simulink model "testing"  (R2025b)
settings: Solver=FixedStepDiscrete  StartTime=0.0  StopTime=20  RelTol=1e-3
InitFcn:
  | mcb_pmsm_foc_qep_f28379d_SIUnit_data
values from neighbouring files (symbols this model uses):
  A = [ -Rs/L,           0,                  0 ... (first row only)    [mcb_pmsm_fsfb_f28379d_param.m]    (also in v0_pmsm_fsfb_sim_for_flipsky_.m = [; v1_0_3_sim_param_fsfc.m = [)
  inverter = mcb.updateInverterParameters(pmsm,inverter,target)    [mcb_pmsm_foc_qep_f28379d_SIUnit_data.m]
  K = Ka_fsfb(1)    [mcb_pmsm_foc_qep_f28379d_SIUnit_data.m]    (also in mcb_pmsm_fsfb_f28379d_param.m = place(Ai, Bi, desired_poles); v0_pmsm_fsfb_sim_for_flipsky_.m = place(Ai, Bi, desired_poles); v1_0_3_sim_param_fsfc.m = place(Ai, Bi, desired_poles))
  Ki = -Ka_fsfb(2)    [mcb_pmsm_foc_qep_f28379d_SIUnit_data.m]    (also in mcb_pmsm_fsfb_f28379d_param.m = -K(:, n+1:end); v0_pmsm_fsfb_sim_for_flipsky_.m = -K(:, n+1:end); v1_0_3_sim_param_fsfc.m = -K(:, n+1:end))
  lambda_pm = pmsm.FluxPM    [mcb_pmsm_foc_qep_f28379d_SIUnit_data.m]
  PI_params = mcb.calcFOCGains(motor,Ts,Ts_speed,SpdLPFltCoeff=LPFltCoeff)    [mcb_pmsm_foc_qep_f28379d_SIUnit_data.m]
  pmsm = mcb.getPMSMParameters('Teknic2310P')    [mcb_pmsm_foc_qep_f28379d_SIUnit_data.m]
  Speed_Ki_Ts = Kis * Ts_speed    [mcb_pmsm_foc_qep_f28379d_SIUnit_data.m]
  Speed_Kp = Ks    [mcb_pmsm_foc_qep_f28379d_SIUnit_data.m]
  T_pwm = 1/PWM_frequency    (= 5e-05)    [mcb_pmsm_foc_qep_f28379d_SIUnit_data.m]
  target = mcb.getProcessorParameters('F28379D',PWM_frequency)    [mcb_pmsm_foc_qep_f28379d_SIUnit_data.m]
  Ts = T_pwm    (= 5e-05)    [mcb_pmsm_foc_qep_f28379d_SIUnit_data.m]    (also in v0_pmsm_fsfb_sim_for_flipsky_.m = 0.0001; v1_0_3_sim_param_fsfc.m = 0.0001)
  Ts_inverter = T_pwm/2    (= 2.5e-05)    [mcb_pmsm_foc_qep_f28379d_SIUnit_data.m]
  Ts_motor = T_pwm/2    (= 2.5e-05)    [mcb_pmsm_foc_qep_f28379d_SIUnit_data.m]
  Ts_simulink = T_pwm/2    (= 2.5e-05)    [mcb_pmsm_foc_qep_f28379d_SIUnit_data.m]
  Ts_speed = 10*Ts    (= 0.0005)    [mcb_pmsm_foc_qep_f28379d_SIUnit_data.m]
undefined symbols (not defined in the file or in its folder): bit, DiscIntNeverNeededParam, Down, GPTRIP1SEL, GPTRIP2SEL, TZ1, TZ2, Up
libraries: mcbcontrolslib x10, c2802xlib x7, simulink x5, c2837xDlib x4, mcbeeMathTransformLib x3, c280xlib x3, mcbpositiondecoderlib x3, svdschedulerlib x1, autolibpmsmexterior x1, slpidlib x1
(part 1 of 2)
settings Model: SimulationMode=external  ExtModeTrigDuration=8  Creator=LabPC  LastModifiedBy=LabPC
settings OptimizationCC: DefaultUnderspecifiedDataType=single  EnhancedBackFolding=on  PassReuseOutputArgsAs=Individual arguments  MaxStackSize=1024  OptimizeBlockOrder=speed  DifferentSizesBufferReuse=on  OptimizationCustomize=off  EfficientTunableParamExpr=on
settings DebuggingCC: MultiTaskDSMMsg=none  ParameterTunabilityLossMsg=error
settings HardwareCC: ProdBitPerChar=16.0  ProdBitPerInt=16.0  ProdBitPerPointer=32.0  ProdBitPerSizeT=32.0  ProdBitPerPtrDiffT=32.0  ProdLargestAtomicInteger=Integer  ProdLargestAtomicFloat=None  ProdWordSize=16.0  ProdLongLongMode=on  ProdHWDeviceType=Texas Instruments->C2000  HardwareBoardFeatureSet=SoCBlockset
settings SFSimCC: MATLABDynamicMemAlloc=off
settings RTWCC: SystemTargetFile=ert.tlc  HardwareBoard=TI Delfino F28379D LaunchPad  TLCOptions="-aInlineSetEventsForThisBaseRateFcn=TLC_FALSE -aSuppressMultiTaskScheduler=TLC_FALSE   -aRateBasedStepFcn=1"  TemplateMakefile=ert_default_tmf  Toolchain=Texas Instruments Code Composer Studio (C2000)  BuildConfiguration=Faster Runs  CodeProfilingSaveOptions=MetricsOnly  Description=Embedded Coder
settings CodeAppCC: ForceParamTrailComments=on  IgnoreCustomStorageClasses=off  OperatorAnnotations=on  SimulinkDataObjDesc=on  SFDataObjDesc=on  InsertBlockDesc=on
settings ERTTargetCC: ExtModeTransport=4.0  ExtModeStaticAlloc=on  ExtModeAutomaticAllocSize=off  ExtModeStaticAllocSize=10000.0  ExtModeMexFile=ext_xcp  ExtModeIntrfLevel=Level2 - Open  InlinedParameterPlacement=Hierarchical  CodeReplacementLibrary=TI C28x  SupportContinuousTime=on

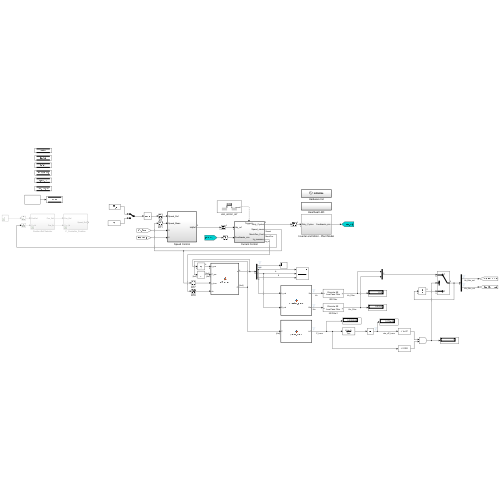
[thumbnail: Simulink's stored preview of the top-level diagram]
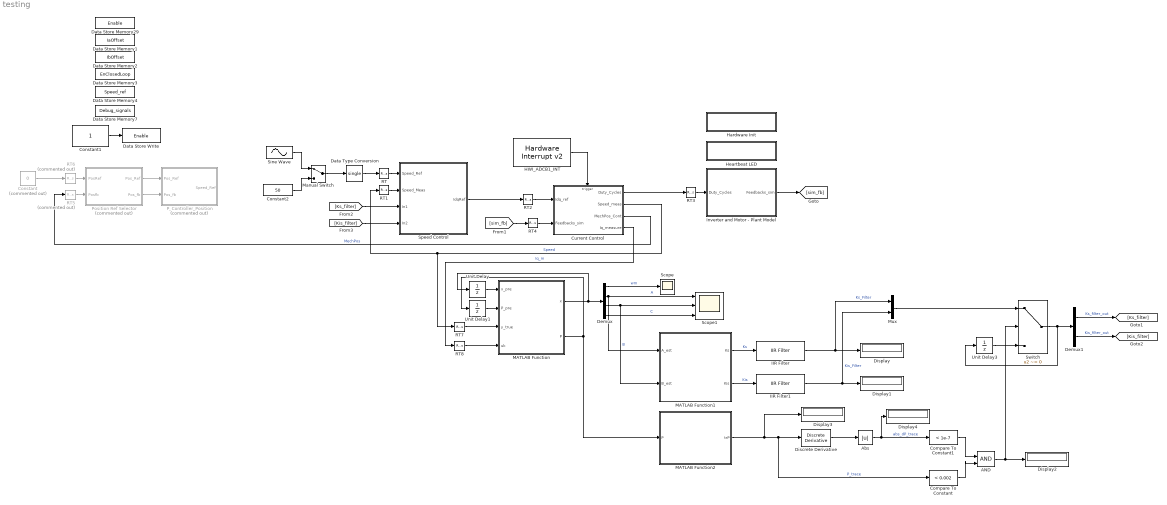
== system testing ==
  AND : Logic  IconShape=distinctive  AllPortsSameDT=off  OutDataTypeStr=boolean
  Abs : Abs  SaturateOnIntegerOverflow=off
  Compare To Constant : simulink/Logic and Bit Operations/Compare To Constant  relop=<  const=0.002  OutDataTypeStr=boolean
  Compare To Constant1 : simulink/Logic and Bit Operations/Compare To Constant  relop=<  const=1e-7  OutDataTypeStr=boolean
  Constant : Constant  Commented=on  Value=0
  Constant1 : Constant  OutDataTypeStr=boolean
  Constant2 : Constant  Value=50
  Current Control : Subsystem
      settings: RTWSystemCode=Nonreusable function
  Data Store Memory1 : DataStoreMemory  DataStoreName=IaOffset  InitialValue=inverter.CtSensAOffset  ShowAdditionalParam=off
  Data Store Memory2 : DataStoreMemory  DataStoreName=IbOffset  InitialValue=inverter.CtSensBOffset  ShowAdditionalParam=off
  Data Store Memory29 : DataStoreMemory  DataStoreName=Enable  ShowAdditionalParam=off  OutDataTypeStr=boolean
  Data Store Memory3 : DataStoreMemory  DataStoreName=EnClosedLoop  ShowAdditionalParam=off  OutDataTypeStr=boolean
  Data Store Memory4 : DataStoreMemory  DataStoreName=Speed_ref  ShowAdditionalParam=off  OutDataTypeStr=dataType
  Data Store Memory7 : DataStoreMemory  DataStoreName=Debug_signals  InitialValue=5  ShowAdditionalParam=off  OutDataTypeStr=uint16
  Data Store Write : DataStoreWrite  DataStoreName=Enable  IndexOptions=Index vector (dialog)  Indices=1  OutputSizes=1
  Data Type Conversion : DataTypeConversion  OutDataTypeStr=single  SaturateOnIntegerOverflow=off  RndMeth=Floor
  Demux : Demux
  Demux1 : Demux  Outputs=2
  Discrete Derivative : simulink/Discrete/Discrete Derivative  gainval=1.0  ICPrevScaledInput=10  OutMin=[]  OutMax=[]  OutDataType=fixdt(1, 16)  OutScaling=2^-10  DoSatur=off
  Display{,1..4} (5 alike) : Display
  HWI_ADCB1_INT : svdschedulerlib/Hardware Interrupt v2  ISRGroup=ADC - Analog to Digital Converter  ISRName=ADCA1_INT  ISRNumber=32  NumEventsToServe=1  EventsList={'on','EOC event','1';'off','Overflow event','2';'off','Custom event','3'}  SelectedEvents={'event1'}  TaskPriority=30  DisablePreemption=off  ClearInterruptFlagsAtEndOfEvent=on  InterruptDefinitionFile=$(TARGET_ROOT)/registry/interrupts/F2837xS_interrupts.xml  HardwareBoard=F2837x  EnableSimPort=off
      settings: LibrarySourceBlock=c2000lib/Scheduling/Hardware Interrupt
  Hardware Init : Subsystem  TreatAsAtomicUnit=on
  Heartbeat LED : Subsystem  TreatAsAtomicUnit=on
  IIR Filter : mcbcontrolslib/IIR Filter  VariantControl=Low Pass Filter  VariantSelect=Low-pass  FilterConstantInputType=Specify via dialog  Filter_constant=0.001  InitialOutput=Specify via dialog  InitialOutputValue=0  ExternalReset=none  advancedSettings=off  Ts=50e-6  cutOff_freq=3.1863
  IIR Filter1 : mcbcontrolslib/IIR Filter  VariantControl=Low Pass Filter  VariantSelect=Low-pass  FilterConstantInputType=Specify via dialog  Filter_constant=0.001  InitialOutput=Specify via dialog  InitialOutputValue=0  ExternalReset=none  advancedSettings=off  Ts=50e-6  cutOff_freq=3.1863
  Inverter and Motor - Plant Model : Subsystem
  MATLAB Function : MATLAB Function  TreatAsAtomicUnit=on
  MATLAB Function1 : MATLAB Function  TreatAsAtomicUnit=on
  MATLAB Function2 : MATLAB Function  TreatAsAtomicUnit=on
  Manual Switch : ManualSwitch
  Mux : Mux  Inputs=2
  P_Controller_Position : Subsystem  Commented=on
  Position Ref Selector : Subsystem  Commented=on
  RT{,1,7..8} (4 alike) : RateTransition  Deterministic=off  OutPortSampleTime=Ts_speed
  RT2 : RateTransition  Deterministic=off
  RT3 : RateTransition  Deterministic=off
  RT4 : RateTransition  Deterministic=off
  RT5 : RateTransition  Commented=on  Deterministic=off  OutPortSampleTime=Ts_speed
  RT6 : RateTransition  Commented=on  Deterministic=off  OutPortSampleTime=Ts_speed
  Scope : Scope
      settings: ActiveDisplayYMinimum=-2525.7371063232422  ActiveDisplayYMaximum=2611.2176971435547
  Scope1 : Scope  NumInputPorts=3
      settings: ActiveDisplayYMinimum=-2525.7371063232422  ActiveDisplayYMaximum=2611.2176971435547
  Sine Wave : Sin  Amplitude=100  Frequency=5  SampleTime=Ts_speed
  Speed Control : Subsystem  TreatAsAtomicUnit=on  SystemSampleTime=Ts_speed
  Switch : Switch  Criteria=u2 ~= 0  SaturateOnIntegerOverflow=off  InputSameDT=off
  Unit Delay : UnitDelay  InitialCondition=[0; 0.3734; 5438; 0.1]  SampleTime=-1  HasFrameUpgradeWarning=on
  Unit Delay1 : UnitDelay  InitialCondition=diag([1 10 10 100])  SampleTime=-1  HasFrameUpgradeWarning=on
  Unit Delay3 : UnitDelay  InitialCondition=[0.0202, 2.7604e-04]  SampleTime=-1  HasFrameUpgradeWarning=on
  wires:
  RT4/1 -> Current Control/2(Feedbacks_sim)
  Speed Control/1(IdqRef) -> RT2/1
  Inverter and Motor - Plant Model/1(Feedbacks_sim) -> [sim_fb]
  Current Control/1(Duty_Cycles) -> RT3/1
  Current Control/2(Speed_meas) -> RT1/1, RT7/1  "Speed"
  RT/1 -> Speed Control/1(Speed_Ref)
  RT2/1 -> Current Control/1(Idq_ref)
  RT1/1 -> Speed Control/2(Speed_Meas)
  RT3/1 -> Inverter and Motor - Plant Model/1(Duty_Cycles)
  [sim_fb] -> RT4/1
  Constant1/1 -> Data Store Write/1
  HWI_ADCB1_INT/1 -> Current Control/Trigger
  Constant/1 -> RT6/1
  Position Ref Selector/1(Pos_Ref) -> P_Controller_Position/1(Pos_Ref)
  Position Ref Selector/2(Pos_fb) -> P_Controller_Position/2(Pos_fb)
  Current Control/3(MechPos_Cont) -> RT5/1  "MechPos"
  RT5/1 -> Position Ref Selector/2(Posfb)
  RT6/1 -> Position Ref Selector/1(PosRef)
  MATLAB Function/1(x) -> Demux/1, Unit Delay/1
  Unit Delay/1 -> MATLAB Function/1(x_pre)
  Unit Delay1/1 -> MATLAB Function/2(P_pre)
  MATLAB Function/2(P) -> MATLAB Function2/1(P), Unit Delay1/1
  RT7/1 -> MATLAB Function/3(y_true)
  Current Control/4(Iq_measure) -> RT8/1  "Iq_m"
  RT8/1 -> MATLAB Function/4(uk)
  Demux/3 -> MATLAB Function1/2(B_est), Scope1/2  "B"
  Demux/2 -> MATLAB Function1/1(A_est), Scope1/1  "A"
  Data Type Conversion/1 -> RT/1
  MATLAB Function1/1(Ks) -> IIR Filter/1  "Ks"
  IIR Filter/1 -> Mux/1, Display/1  "Ks_Filter"
  MATLAB Function1/2(Kis) -> IIR Filter1/1  "Kis"
  IIR Filter1/1 -> Mux/2, Display1/1  "Kis_Filter"
  Manual Switch/1 -> Data Type Conversion/1
  Sine Wave/1 -> Manual Switch/1
  Constant2/1 -> Manual Switch/2
  MATLAB Function2/1(trP) -> Display3/1, Discrete Derivative/1, Compare To Constant/1  "P_trace"
  Discrete Derivative/1 -> Abs/1
  Abs/1 -> Display4/1, Compare To Constant1/1  "abs_dP_trace"
  Compare To Constant1/1 -> AND/1
  Compare To Constant/1 -> AND/2
  AND/1 -> Display2/1, Switch/2
  Mux/1 -> Switch/1
  Unit Delay3/1 -> Switch/3
  Switch/1 -> Unit Delay3/1, Demux1/1
  Demux1/1 -> [Ks_filter]  "Ks_filter_out"
  Demux1/2 -> [Kis_filter]  "Kis_filter_out"
  [Ks_filter] -> Speed Control/3(In1)
  [Kis_filter] -> Speed Control/4(In2)
  Demux/1 -> Scope/1  "wm"
  Demux/4 -> Scope1/3  "C"

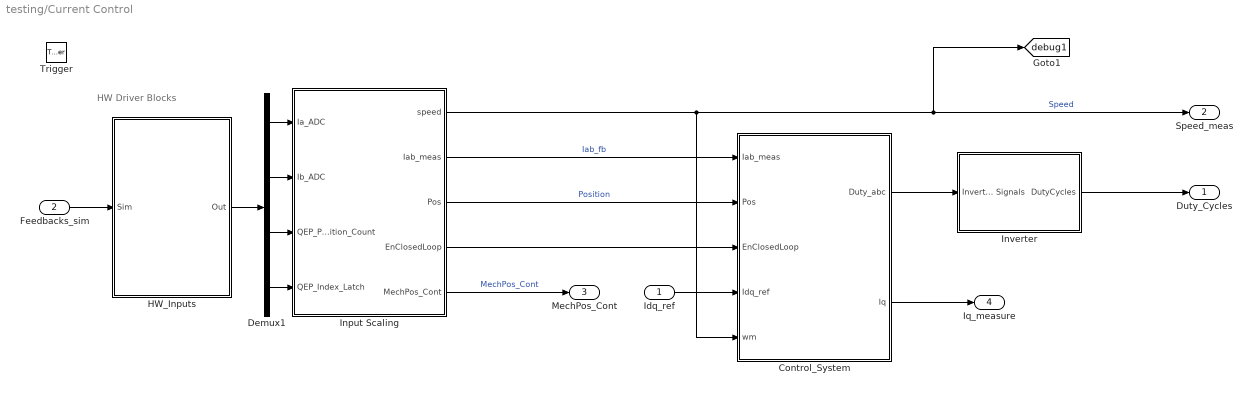
== system testing/Current Control ==
  note: HW Driver Blocks
  Idq_ref : Inport
  Feedbacks_sim : Inport  Port=2
  Trigger : TriggerPort  TriggerType=function-call  VariantControl=Variant  PortDimensions=1
  Control_System : Subsystem  TreatAsAtomicUnit=on
  Demux1 : Demux
  HW_Inputs : Subsystem  Variant=on  VariantControlMode=sim codegen switching
  Input Scaling : Subsystem
  Inverter : Subsystem  Variant=on  VariantControlMode=sim codegen switching
  Duty_Cycles : Outport  InitialOutput=0  VectorParamsAs1DForOutWhenUnconnected=off
  Speed_meas : Outport  Port=2  InitialOutput=0  VectorParamsAs1DForOutWhenUnconnected=off
  MechPos_Cont : Outport  Port=3  InitialOutput=0  VectorParamsAs1DForOutWhenUnconnected=off
  Iq_measure : Outport  Port=4  InitialOutput=0  VectorParamsAs1DForOutWhenUnconnected=off
  tag scope: debug1=global
  wires:
  Input Scaling/3(Pos) -> Control_System/2(Pos)  "Position"
  Idq_ref/1 -> Control_System/4(Idq_ref)
  Input Scaling/1(speed) -> Control_System/5(wm), Speed_meas/1, [debug1]  "Speed"
  Input Scaling/2(Iab_meas) -> Control_System/1(Iab_meas)  "Iab_fb"
  Demux1/1 -> Input Scaling/1(Ia_ADC)
  Demux1/2 -> Input Scaling/2(Ib_ADC)
  Demux1/3 -> Input Scaling/3(QEP_Position_Count)
  Demux1/4 -> Input Scaling/4(QEP_Index_Latch)
  Inverter/1(DutyCycles) -> Duty_Cycles/1
  HW_Inputs/1(Out) -> Demux1/1
  Feedbacks_sim/1 -> HW_Inputs/1(Sim)
  Input Scaling/4(EnClosedLoop) -> Control_System/3(EnClosedLoop)
  Control_System/1(Duty_abc) -> Inverter/1(Inverter Signals)
  Input Scaling/5(MechPos_Cont) -> MechPos_Cont/1  "MechPos_Cont"
  Control_System/2(Iq) -> Iq_measure/1

== system testing/Hardware Init ==
  6PWM_Mode : Constant  Priority=1000  Value=0x3A16  OutDataTypeStr=uint16  SampleTime=-1
  ADC_Gain_Setting : Constant  Priority=1000  Value=inverter.SPI_Gain_Setting  OutDataTypeStr=uint16  SampleTime=-1
  Event Listener : EventListener  DisableCoverage=on  EventName=reset
  Mux : Mux  Inputs=2
  Variant Subsystem : Subsystem  Variant=on  VariantControlMode=sim codegen switching
  wires:
  6PWM_Mode/1 -> Mux/1
  ADC_Gain_Setting/1 -> Mux/2
  Mux/1 -> Variant Subsystem/1(In1)

== system testing/Heartbeat LED ==
  note: Heartbeat LED 1HZ
  Heartbeat LED : Subsystem  Variant=on  VariantControlMode=sim codegen switching
  RED_LED : Constant  OutDataTypeStr=uint16  SampleTime=2
  wires:
  RED_LED/1 -> Heartbeat LED/1(In1)

== system testing/Inverter and Motor - Plant Model ==
  Duty_Cycles : Inport
  Codegeneration : Subsystem
  Simulation : Subsystem
  Variant Sink : VariantSink  VariantControlMode=sim codegen switching  VariantControls={(codegen), (sim)}
  Variant Source1 : VariantSource  VariantControlMode=sim codegen switching  VariantControls={(codegen), (sim)}
  Feedbacks_sim : Outport  VectorParamsAs1DForOutWhenUnconnected=off
  wires:
  Variant Source1/1 -> Feedbacks_sim/1
  Simulation/1(Feedbacks) -> Variant Source1/2
  Codegeneration/1(Feedbacks) -> Variant Source1/1
  Duty_Cycles/1 -> Variant Sink/1
  Variant Sink/2 -> Simulation/1(Duty_Cycles)
  Variant Sink/1 -> Codegeneration/1(Duty_Cycles)

== system testing/P_Controller_Position ==
  Pos_Ref : Inport
  Pos_fb : Inport  Port=2
  Constant : Constant  Value=10  OutDataTypeStr=dataType
  Divide : Product  Inputs=**  OutDataTypeStr=dataType  RndMeth=Simplest
  Saturation : Saturate  UpperLimit=5000  LowerLimit=-5000
  Sum : Sum  Inputs=|+-  OutDataTypeStr=Inherit: Same as first input
  Speed_Ref : Outport
  wires:
  Constant/1 -> Divide/2
  Saturation/1 -> Speed_Ref/1
  Divide/1 -> Saturation/1
  Pos_Ref/1 -> Sum/1
  Pos_fb/1 -> Sum/2
  Sum/1 -> Divide/1  "error_pos"

== system testing/Position Ref Selector ==
  PosRef : Inport
  Posfb : Inport  Port=2
  AND : Logic  IconShape=distinctive  AllPortsSameDT=off  OutDataTypeStr=boolean
  Data Store Read : DataStoreRead  DataStoreName=EnClosedLoop  IndexOptions=Index vector (dialog)  Indices=1  OutputSizes=1
  Data Store Read1 : DataStoreRead  DataStoreName=Enable  IndexOptions=Index vector (dialog)  Indices=1  OutputSizes=1
  Switch : Switch  Criteria=u2 > Threshold  SaturateOnIntegerOverflow=off  InputSameDT=off
  Pos_Ref : Outport
  Pos_fb : Outport  Port=2
  wires:
  Data Store Read/1 -> AND/1
  AND/1 -> Switch/2
  PosRef/1 -> Switch/1
  Data Store Read1/1 -> AND/2
  Switch/1 -> Pos_Ref/1
  Posfb/1 -> Pos_fb/1, Switch/3

== system testing/Speed Control ==
  Speed_Ref : Inport
  Speed_Meas : Inport  Port=2
  In1 : Inport  Port=3
  In2 : Inport  Port=4
  Id_ref : Constant  Value=0  OutDataTypeStr=dataType  SampleTime=Ts_speed
  Mux1 : Mux  Inputs=2
  PI_Controller_Speed : Subsystem
  Subsystem : Subsystem
  IdqRef : Outport  VectorParamsAs1DForOutWhenUnconnected=off
  wires:
  Speed_Meas/1 -> PI_Controller_Speed/2(N_fb), Subsystem/2(Speed_Ref_Open)  "Speed_fb"
  Subsystem/1(Speed_Ref_PU) -> PI_Controller_Speed/1(N_ref)  "Speed_Ref"
  Id_ref/1 -> Mux1/1
  PI_Controller_Speed/1(Iq_ref) -> Mux1/2
  Mux1/1 -> IdqRef/1
  Speed_Ref/1 -> Subsystem/1(Speed_Ref_In)
  In1/1 -> PI_Controller_Speed/3(In1)  "Ks_filter"
  In2/1 -> PI_Controller_Speed/4(In2)  "Kis_filter"

== system testing/Current Control/Control_System ==
  Iab_meas : Inport
  Pos : Inport  Port=2
  EnClosedLoop : Inport  Port=3
  Idq_ref : Inport  Port=4
  wm : Inport  Port=5
  Closed Loop Control : Subsystem
  NOT : Logic  Operator=NOT  IconShape=distinctive  AllPortsSameDT=off  OutDataTypeStr=boolean
  Open Loop Start-Up : Subsystem
  Switch4 : Switch  Threshold=0.5  OutDataTypeStr=Inherit: Inherit via back propagation  RndMeth=Simplest  SaturateOnIntegerOverflow=off  InputSameDT=off
  Duty_abc : Outport  VectorParamsAs1DForOutWhenUnconnected=off
  Iq : Outport  Port=2  VectorParamsAs1DForOutWhenUnconnected=off
  wires:
  EnClosedLoop/1 -> NOT/1, Switch4/2, Closed Loop Control/Enable
  Open Loop Start-Up/1(Duty_abc) -> Switch4/3
  Iab_meas/1 -> Closed Loop Control/1(Iab_meas)
  Pos/1 -> Closed Loop Control/2(Pos)
  Idq_ref/1 -> Closed Loop Control/3(Idq_ref)
  Closed Loop Control/2(Duty_abc) -> Switch4/1
  NOT/1 -> Open Loop Start-Up/Enable
  Switch4/1 -> Duty_abc/1  "PWM_Duty_Cycles"
  Closed Loop Control/1(Iq) -> Iq/1
  wm/1 -> Closed Loop Control/4(wm)

== system testing/Current Control/HW_Inputs ==
  Sim : Inport
  Sensor Driver Blocks (codegen) : Subsystem  VariantControl=(codegen)
  Sensor Driver Blocks (sim) : Subsystem  VariantControl=(sim)
  Out : Outport

== system testing/Current Control/Input Scaling ==
  note: Current Measurements
  note: Position & Speed Measurements
  note: QEP
  Ia_ADC : Inport
  Ib_ADC : Inport  Port=2
  QEP_Position_Count : Inport  Port=3
  QEP_Index_Latch : Inport  Port=4
  " Calculate Position and Speed" : Subsystem
  Calculate Phase Currents : Subsystem
  IndexOffset : Constant  Value=pmsm.PositionOffset * 2 * pi  OutDataTypeStr=dataType  SampleTime=-1
  speed : Outport
  Iab_meas : Outport  Port=2
  Pos : Outport  Port=3
  EnClosedLoop : Outport  Port=4
  MechPos_Cont : Outport  Port=5
  wires:
  " Calculate Position and Speed"/2(speed) -> speed/1
  Calculate Phase Currents/1(Iab_meas) -> Iab_meas/1  "Iab_fb"
  QEP_Position_Count/1 -> " Calculate Position and Speed"/1(QEP_Position_Count)
  " Calculate Position and Speed"/1(Theta_e) -> Pos/1
  Ia_ADC/1 -> Calculate Phase Currents/1(Ia_ADC)
  Ib_ADC/1 -> Calculate Phase Currents/2(Ib_ADC)
  QEP_Index_Latch/1 -> " Calculate Position and Speed"/2(QEP_Index_Latch)
  IndexOffset/1 -> " Calculate Position and Speed"/3(Offset)
  " Calculate Position and Speed"/3(IndexFound) -> EnClosedLoop/1
  " Calculate Position and Speed"/4(MechPos_Cont) -> MechPos_Cont/1

== system testing/Current Control/Inverter ==
  Inverter Signals : Inport
  Code Generation : Subsystem  VariantControl=(codegen)
  Simulation : Subsystem  VariantControl=(sim)
  DutyCycles : Outport  VectorParamsAs1DForOutWhenUnconnected=off

== system testing/Hardware Init/Variant Subsystem ==
  In1 : Inport
  Code Generation : Subsystem  VariantControl=(codegen)
  Simulation : Subsystem  VariantControl=(sim)

== system testing/Heartbeat LED/Heartbeat LED ==
  In1 : Inport
  Code generation : Subsystem  VariantControl=(codegen)
  Simulation : Subsystem  VariantControl=(sim)

== system testing/Inverter and Motor - Plant Model/Codegeneration ==
  Duty_Cycles : Inport
  Ground : Ground
  Terminator : Terminator
  Feedbacks : Outport  VectorParamsAs1DForOutWhenUnconnected=off
  wires:
  Duty_Cycles/1 -> Terminator/1
  Ground/1 -> Feedbacks/1

== system testing/Inverter and Motor - Plant Model/Simulation ==
  Duty_Cycles : Inport
  Inverter : Subsystem
  Load_Profile (Torque) : Subsystem
  RT1 : RateTransition  Deterministic=off  OutPortSampleTime=Ts_simulink
  RT3 : RateTransition  Deterministic=off  OutPortSampleTime=Ts_simulink
  Rate Transition : RateTransition  Integrity=off  OutPortSampleTime=Ts_motor
  Rate Transition1 : RateTransition  Integrity=off  OutPortSampleTime=Ts_motor
  Sensor_Measurements : Subsystem
  Surface Mount PMSM : autolibpmsmexterior/Surface Mount PMSM  port_config=Torque  sim_type=Discrete  Ts=Ts_motor  P=pmsm.p  Rs=pmsm.Rs + inverter.R_board  Ldq_=pmsm.Ld  KConstText=Permanent flux linkage constant (lambda_pm):  lambda_pm=pmsm.FluxPM  Ke=159.9771  Kt=1.323  mechanical=[pmsm.J, pmsm.B, 0]  idq0=[0 0]  theta_init=0  omega_init=0  KConst=pmsm.FluxPM  lambda_pm_calc=pmsm.FluxPM  RefBlkName='autolibpmsmexterior/Surface Mount PMSM'  aMode=5  Ldq="[0.00105     0.00105]"
  Terminator : Terminator
  Feedbacks : Outport  VectorParamsAs1DForOutWhenUnconnected=off
  wires:
  Rate Transition1/1 -> Surface Mount PMSM/1
  Surface Mount PMSM/2 -> RT1/1  "Iabc"
  Surface Mount PMSM/3 -> Terminator/1
  Rate Transition/1 -> Surface Mount PMSM/2  "PhaseVoltage"
  RT1/1 -> Sensor_Measurements/2(PhaseCurr)
  Duty_Cycles/1 -> Inverter/1(Duty_abc)
  Inverter/1(Vabc) -> Rate Transition/1
  RT3/1 -> Sensor_Measurements/1(Info)
  Surface Mount PMSM/1 -> RT3/1
  Load_Profile (Torque)/1(Load_Trq) -> Rate Transition1/1
  Sensor_Measurements/1(Sim_fb) -> Feedbacks/1

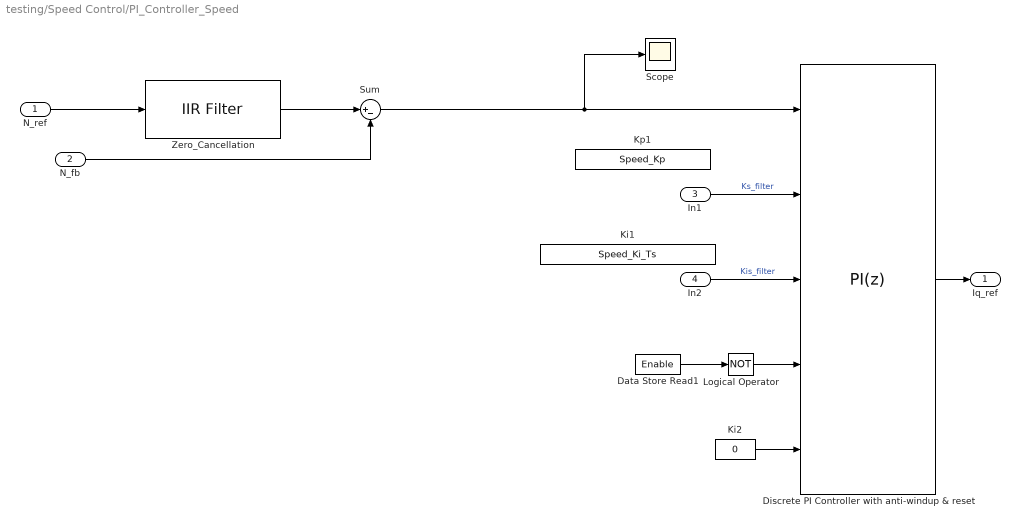
== system testing/Speed Control/PI_Controller_Speed ==
  N_ref : Inport
  N_fb : Inport  Port=2
  In1 : Inport  Port=3
  In2 : Inport  Port=4
  Data Store Read1 : DataStoreRead  DataStoreName=Enable  IndexOptions=Index vector (dialog)  Indices=1  OutputSizes=1
  Discrete PI Controller with anti-windup & reset : slpidlib/PID Controller  Controller=PI  Form=Parallel  TimeDomain=Discrete-time  UseExternalTs=off  SampleTime=-1  IntegratorMethod=Forward Euler  FilterMethod=Forward Euler  ControllerParametersSource=external  P=1  I=1  UseKiTs=on  D=0  UseExternalDerivativeSource=off  N=100  UseFilter=on  TunerSelectOption=Transfer Function Based (PID Tuner App)  InitialConditionSource=external  InitialConditionForIntegrator=0  InitialConditionForFilter=0  DifferentiatorICPrevScaledInput=0  ExternalReset=level  TrackingMode=off  Kt=1  LimitOutput=on  SatLimitsSource=internal  UpperSaturationLimit=inverter.ISenseMax  LowerSaturationLimit=-inverter.ISenseMax  LinearizeAsGain=on  AntiWindupMode=clamping  Kb=1  LimitIntegrator=off  UpperIntegratorSaturationLimit=inf  LowerIntegratorSaturationLimit=-inf  RndMeth=Simplest  POutMin=[]  POutMax=[]  IOutMin=[]  IOutMax=[]  DOutMin=[]  DOutMax=[]  NOutMin=[]  NOutMax=[]  SumOutMin=[]  SumOutMax=[]  SaturationOutDataTypeStr=Inherit: Inherit via back propagation  SaturationOutMin=[]  SaturationOutMax=[]  PParamMin=[]  PParamMax=[]  IParamMin=[]  IParamMax=[]  DParamMin=[]  DParamMax=[]  NParamMin=[]  NParamMax=[]  KbParamMin=[]  KbParamMax=[]  KtParamMin=[]  KtParamMax=[]  KbOutMin=[]  KbOutMax=[]  KtOutMin=[]  KtOutMax=[]  IntegratorOutMin=[]  IntegratorOutMax=[]  FilterOutMin=[]  FilterOutMax=[]  SumI1OutMin=[]  SumI1OutMax=[]  SumI2OutMin=[]  SumI2OutMax=[]  SumI3OutMin=[]  SumI3OutMax=[]  SumI4OutMin=[]  SumI4OutMax=[]  SumDOutMin=[]  SumDOutMax=[]  DifferentiatorOutMin=[]  DifferentiatorOutMax=[]  FilterDiffOutCoefMin=[]  FilterDiffOutCoefMax=[]  ReciprocalOutMin=[]  ReciprocalOutMax=[]  SumDenOutMin=[]  SumDenOutMax=[]  SumNumOutMin=[]  SumNumOutMax=[]  DivideOutMin=[]  DivideOutMax=[]  UdiffTsProdOutMin=[]  UdiffTsProdOutMax=[]  NTsProdOutMin=[]  NTsProdOutMax=[]  UintegralTsProdOutMin=[]  UintegralTsProdOutMax=[]  UngainTsProdOutMin=[]  UngainTsProdOutMax=[]  ClampingZeroOutDataTypeStr=Inherit: Inherit via back propagation  ClampingZeroOutMin=[]  ClampingZeroOutMax=[]  FilterDenConstantOutDataTypeStr=Inherit: Inherit via back propagation  FilterDenConstantOutMin=[]  FilterDenConstantOutMax=[]  PCopyOutDataTypeStr=Inherit: Inherit via back propagation  PCopyOutMin=[]  PCopyOutMax=[]  NCopyOutDataTypeStr=Inherit: Inherit via back propagation  NCopyOutMin=[]  NCopyOutMax=[]  IntegratorContinuousStateAttributes=''  IntegratorStateMustResolveToSignalObject=off  IntegratorRTWStateStorageClass=Auto  FilterContinuousStateAttributes=''  FilterStateMustResolveToSignalObject=off  FilterRTWStateStorageClass=Auto  ParallelPVariant=ExternalParameters  IdealPVariant=Disabled  IVariant=ExternalParameters  DVariant=Disabled  IntegratorVariant=Discrete  SatVariant=Enabled  AWVariant=DiscClampingParallel  PCopyVariant=Disabled  TRVariant=Disabled  FdbkBlocksVariant=Forward  IdealPFdbkVariant=Disabled  SatFdbkVariant=Disabled  DerivativeFilterVariant=Disabled  NVariant=Disabled  NCopyVariant=Disabled_SignalSpec  FilterICVariant=Disabled  IntegratorICVariant=ExternalICs  ExternalResetVariant=ExternalReset  TRSumVariant=Passthrough  SumFdbkVariant=Disabled  SumVariant=Sum_PI  TsampFilterVariant=InternalTs  TsampNgainVariant=Passthrough  TsampIntegralVariant=Disabled_SignalSpec  ExternalSaturationOutDataTypeStr=Inherit: Same as second input  DerivativeSourceVariant=Disabled  PreIntVariant=InternalPreInt
      settings: LibrarySourceBlock=mcbcontrolslib/PI Controller
  Ki1 : Constant  Value=Speed_Ki_Ts  OutDataTypeStr=dataType  SampleTime=-1
  Ki2 : Constant  Value=0  OutDataTypeStr=dataType  SampleTime=-1
  Kp1 : Constant  Value=Speed_Kp  OutDataTypeStr=dataType  SampleTime=-1
  Logical Operator : Logic  Operator=NOT  IconShape=distinctive  AllPortsSameDT=off  OutDataTypeStr=boolean
  Scope : Scope
      settings: ActiveDisplayYMinimum=-12.100083367889781  ActiveDisplayYMaximum=11.106556656295403  DataLoggingVariableName=ScopeData7
  Sum : Sum  Inputs=|+-  OutDataTypeStr=Inherit: Same as first input
  Zero_Cancellation : mcbcontrolslib/IIR Filter  VariantControl=Low Pass Filter  VariantSelect=Low-pass  FilterConstantInputType=Specify via dialog  Filter_constant=0.01*(Ts_speed/Ts)  InitialOutput=Specify via dialog  InitialOutputValue=0  ExternalReset=none  advancedSettings=off  Ts=50e-6  cutOff_freq=353.6777
  Iq_ref : Outport  VectorParamsAs1DForOutWhenUnconnected=off
  wires:
  Discrete PI Controller with anti-windup & reset/1 -> Iq_ref/1
  Sum/1 -> Scope/1, Discrete PI Controller with anti-windup & reset/1
  Logical Operator/1 -> Discrete PI Controller with anti-windup & reset/4
  Ki2/1 -> Discrete PI Controller with anti-windup & reset/5
  Data Store Read1/1 -> Logical Operator/1
  N_ref/1 -> Zero_Cancellation/1
  N_fb/1 -> Sum/2
  Zero_Cancellation/1 -> Sum/1
  In1/1 -> Discrete PI Controller with anti-windup & reset/2  "Ks_filter"
  In2/1 -> Discrete PI Controller with anti-windup & reset/3  "Kis_filter"

== system testing/Speed Control/Subsystem ==
  Speed_Ref_In : Inport
  Speed_Ref_Open : Inport  Port=2
  AND : Logic  IconShape=distinctive  AllPortsSameDT=off  OutDataTypeStr=boolean
  Data Store Read : DataStoreRead  DataStoreName=EnClosedLoop  IndexOptions=Index vector (dialog)  Indices=1  OutputSizes=1
  Data Store Read1 : DataStoreRead  DataStoreName=Enable  IndexOptions=Index vector (dialog)  Indices=1  OutputSizes=1
  Switch : Switch  Criteria=u2 > Threshold  Threshold=0.5  SaturateOnIntegerOverflow=off  InputSameDT=off
  Speed_Ref_PU : Outport
  wires:
  Switch/1 -> Speed_Ref_PU/1
  Speed_Ref_Open/1 -> Switch/3
  Speed_Ref_In/1 -> Switch/1
  AND/1 -> Switch/2
  Data Store Read/1 -> AND/1
  Data Store Read1/1 -> AND/2

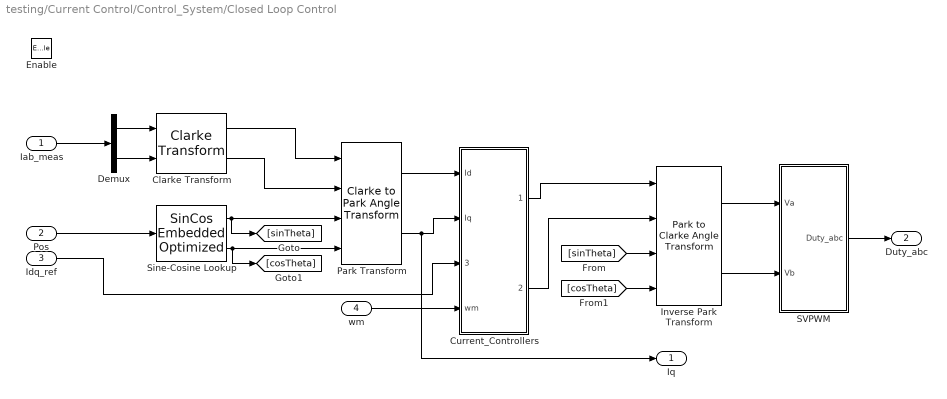
== system testing/Current Control/Control_System/Closed Loop Control ==
  Iab_meas : Inport
  Pos : Inport  Port=2
  Idq_ref : Inport  Port=3
  wm : Inport  Port=4
  Enable : EnablePort  StatesWhenEnabling=reset
  Clarke Transform : mcbeeMathTransformLib/Clarke Transform  VariantControl=Variant2  PowerInvariant=off  UseWithEmbedded=on  PhaseInput=Two inputs
      settings: LibrarySourceBlock=mcbcontrolslib/Clarke Transform
  Current_Controllers : Subsystem
  Demux : Demux  Outputs=2
  Inverse Park Transform : mcbeeMathTransformLib/Park to Clarke Angle Transform  AxisAlignment=D-axis  UseWithEmbedded=on  PhaseInput=Two inputs  ThetaInput=Sine and Cosine electrical position  AngleInput=Per-unit  N_points=1024
      settings: LibrarySourceBlock=mcbcontrolslib/Inverse Park Transform
  Park Transform : mcbeeMathTransformLib/Clarke to Park Angle Transform  AxisAlignment=D-axis  UseWithEmbedded=on  PhaseInput=Two inputs  ThetaInput=Sine and Cosine electrical position  AngleInput=Per-unit  N_points=1024
      settings: LibrarySourceBlock=mcbcontrolslib/Park Transform
  SVPWM : Subsystem
  Sine-Cosine Lookup : mcbcontrolslib/SinCos Embedded Optimized  LabelModeActiveChoice=MCB_Sin  OptforProc=off  ApproximationMethod=None  UserApproxMethod=Lookup  ApproxStatus=None  InterpMethod=Linear point-slope  NumberOfDataPoints=16  NumberOfIterations=11  RemoveProtectionAgainstOutOfRangeInput=off  TableDataTypeStr=Inherit: Inherit via input  AngleInput=Radians  ThetaDataType=single  N_points=1024  DatatypeInput=Inherit from input  Datatype=Inherit: Same as input
  Iq : Outport  VectorParamsAs1DForOutWhenUnconnected=off
  Duty_abc : Outport  Port=2  VectorParamsAs1DForOutWhenUnconnected=off
  wires:
  Iab_meas/1 -> Demux/1
  Park Transform/2 -> Current_Controllers/2(Iq), Iq/1
  Park Transform/1 -> Current_Controllers/1(Id)
  Sine-Cosine Lookup/2 -> Park Transform/4, [cosTheta]
  Clarke Transform/1 -> Park Transform/1
  Idq_ref/1 -> Current_Controllers/3(Ida_ref)
  Sine-Cosine Lookup/1 -> [sinTheta], Park Transform/3
  Clarke Transform/2 -> Park Transform/2
  [cosTheta] -> Inverse Park Transform/4
  Demux/2 -> Clarke Transform/2
  Pos/1 -> Sine-Cosine Lookup/1
  Demux/1 -> Clarke Transform/1
  [sinTheta] -> Inverse Park Transform/3
  Current_Controllers/1(Vd_ref) -> Inverse Park Transform/1
  Current_Controllers/2(Vq_ref) -> Inverse Park Transform/2
  Inverse Park Transform/1 -> SVPWM/1(Va)
  Inverse Park Transform/2 -> SVPWM/2(Vb)
  SVPWM/1(Duty_abc) -> Duty_abc/1
  wm/1 -> Current_Controllers/4(wm)

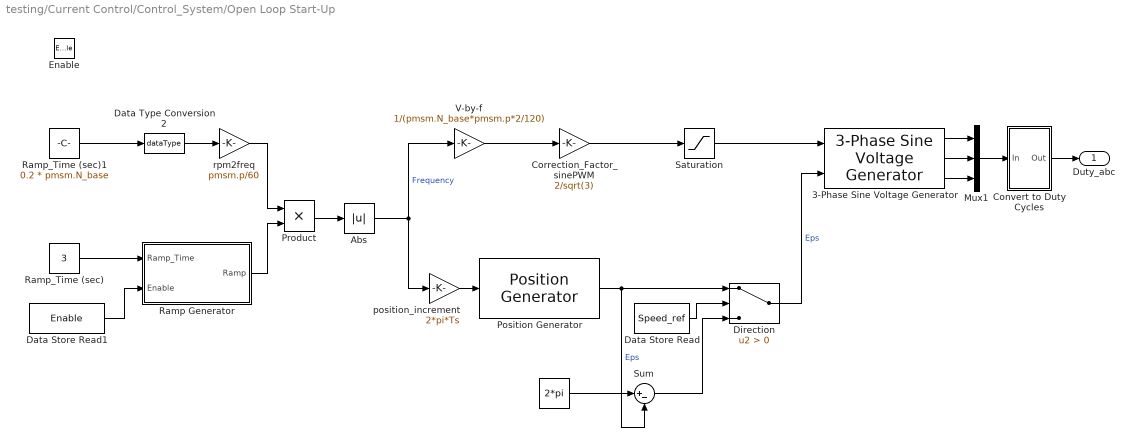
== system testing/Current Control/Control_System/Open Loop Start-Up ==
  Enable : EnablePort  StatesWhenEnabling=reset
  " " : Constant  Value=2*pi  OutDataTypeStr=dataType  SampleTime=-1
  3-Phase Sine Voltage Generator : mcbcontrolslib/3-Phase Sine Voltage Generator  AngleInput=Radians  N_points=1024
  Abs : Abs  SaturateOnIntegerOverflow=off
  Convert to Duty Cycles : Subsystem
  Correction_Factor_sinePWM : Gain  Gain=2/sqrt(3)  RndMeth=Simplest  OutDataTypeStr=Inherit: Same as input
  Data Store Read : DataStoreRead  DataStoreName=Speed_ref  IndexOptions=Index vector (dialog)  Indices=1  OutputSizes=1
  Data Store Read1 : DataStoreRead  DataStoreName=Enable  IndexOptions=Index vector (dialog)  Indices=1  OutputSizes=1
  Data Type Conversion2 : DataTypeConversion  OutDataTypeStr=dataType  RndMeth=Simplest  SaturateOnIntegerOverflow=off
  Direction : Switch  Criteria=u2 > Threshold  OutDataTypeStr=dataType  RndMeth=Simplest  SaturateOnIntegerOverflow=off  InputSameDT=off
  Mux1 : Mux  Inputs=3
  Position Generator : mcbcontrolslib/Position Generator  AngleOutput=Radians  InitialThetaSource=Specify via dialog  ExternalReset=none  Offset=0
  Product : Product  RndMeth=Simplest  OutDataTypeStr=Inherit: Same as first input
  Ramp Generator : Subsystem
  Ramp_Time (sec) : Constant  Value=3  OutDataTypeStr=dataType  SampleTime=-1
  Ramp_Time (sec)1 : Constant  Value=0.2 * pmsm.N_base  OutDataTypeStr=dataType  SampleTime=-1
  Saturation : Saturate  UpperLimit=0.95  LowerLimit=0.15  RndMeth=Simplest
  Sum : Sum  Inputs=|+-  RndMeth=Simplest  OutDataTypeStr=Inherit: Same as first input
  V-by-f : Gain  Gain=1/(pmsm.N_base*pmsm.p*2/120)  RndMeth=Simplest  OutDataTypeStr=Inherit: Same as input
  position_increment : Gain  Gain=2*pi*Ts  RndMeth=Simplest  OutDataTypeStr=Inherit: Same as input
  rpm2freq : Gain  Gain=pmsm.p/60  RndMeth=Simplest  OutDataTypeStr=Inherit: Same as input
  Duty_abc : Outport  VectorParamsAs1DForOutWhenUnconnected=off
  wires:
  3-Phase Sine Voltage Generator/1 -> Mux1/1
  3-Phase Sine Voltage Generator/3 -> Mux1/3
  Direction/1 -> 3-Phase Sine Voltage Generator/2  "Eps"
  Saturation/1 -> 3-Phase Sine Voltage Generator/1
  Ramp Generator/1(Ramp) -> Product/2
  Ramp_Time (sec)/1 -> Ramp Generator/1(Ramp_Time)
  Position Generator/1 -> Sum/2, Direction/1  "Eps"
  " "/1 -> Sum/1
  Sum/1 -> Direction/3
  Abs/1 -> position_increment/1, V-by-f/1  "Frequency"
  position_increment/1 -> Position Generator/1
  V-by-f/1 -> Correction_Factor_sinePWM/1
  Product/1 -> Abs/1
  rpm2freq/1 -> Product/1
  Data Store Read1/1 -> Ramp Generator/2(Enable)
  Correction_Factor_sinePWM/1 -> Saturation/1
  3-Phase Sine Voltage Generator/2 -> Mux1/2
  Data Type Conversion2/1 -> rpm2freq/1
  Ramp_Time (sec)1/1 -> Data Type Conversion2/1
  Data Store Read/1 -> Direction/2
  Mux1/1 -> Convert to Duty Cycles/1(In)
  Convert to Duty Cycles/1(Out) -> Duty_abc/1

== system testing/Current Control/HW_Inputs/Sensor Driver Blocks (codegen) ==
  Sim : Inport
  ADC_B_IN2 : c2802xlib/ADC  blkParamProc=C2000_Type4  ADCModule=B  samplingMode=Single sample mode  ADCResolution=12-bit (Single-ended input)  ADC29xResolution=12-bit  ADCMode=Single-ended input  useSOC1=SOC0  useSOC2=SOC0_SOC1  SOCAcquisitionWindow=15  SOCTriggerSource=ePWM1_ADCSOCA  SOCInterruptTrigger=No ADCINT  Ts=-1  dType=uint16  postInterrupt=on  interruptSel=ADCINT1  ADCINTContinuous=on  endma=off  chdma=1  conv1=ADCINA0  conv2=ADCINA0 and ADCINB0  conv1_Type4=ADCIN2  conv2_Type4=ADCIN0 and ADCIN1
  ADC_C_IN2 : c2802xlib/ADC  blkParamProc=C2000_Type4  ADCModule=C  samplingMode=Single sample mode  ADCResolution=12-bit (Single-ended input)  ADC29xResolution=12-bit  ADCMode=Single-ended input  useSOC1=SOC0  useSOC2=SOC0_SOC1  SOCAcquisitionWindow=15  SOCTriggerSource=ePWM1_ADCSOCA  SOCInterruptTrigger=No ADCINT  Ts=-1  dType=uint16  postInterrupt=off  interruptSel=ADCINT1  ADCINTContinuous=on  endma=off  chdma=1  conv1=ADCINA0  conv2=ADCINA0 and ADCINB0  conv1_Type4=ADCIN2  conv2_Type4=ADCIN0 and ADCIN1
  Mux1 : Mux
  Terminator : Terminator
  eQEP : c280xlib/eQEP  useModule=eQEP1  pcInputmode=Quadrature-count  externalClockrate=2x resolution: Count the rising/falling edge  swapPolarityselection=Clockwise  qdfOutputport=off  qapPolarityselection=on  qbpPolarityselection=on  qipPolarityselection=on  qspPolarityselection=off  igatePolarityselection=off  sampleTime=-1  pcOutputport=on  pcMaximumvalue=2^16-1  indexInitializationcheck=off  indexInitializationevent=Rising edge  strobeInitializationcheck=off  strobeInitializationevent=Rising edge  softwareInitializationcheck=off  softwareInitializationsource=Set to init value at start up  softwareInitializationmode=on  pcInitialvalue=2147483648  pcResetmode=Reset on the first index event  ieloutputport=on  indexEventlatch=Falling edge  seloutputport=off  strobeEventlatch=Rising edge  pcefOutputport=off  enableEqepcapture=off  qctmrOutputport=off  qcprdOutputport=off  captureTimerprescaler=128  upEventprescaler=128  overflowErrorflag=off  directionErrorflag=off  captureTimerposition=On position counter read  unitTimerperiod=100000000  captureTimerlatch=off  capturePeriodlatch=off  positionCounterlatch=off  soenPolarityselection=off  spselPolarityselection=Index pin is used for sync output  compareValuesource=Specify via dialog  shadowMode=Load on QPOSCNT=0  compareValue=4294967295  syncOutputwidth=1  polaritySyncoutput=Active high  watchdogEnable=off  watchdogTimer=65535  outport1Datatype=auto  outport2Datatype=auto  outport3Datatype=auto  outport4Datatype=auto  outport5Datatype=auto  outport6Datatype=auto  outport7Datatype=auto  outport8Datatype=auto  outport9Datatype=auto  outport10Datatype=auto  outport11Datatype=auto  outport12Datatype=auto  eqepinterrupt_pce=off  eqepinterrupt_qpe=off  eqepinterrupt_qdc=off  eqepinterrupt_wto=off  eqepinterrupt_pcu=off  eqepinterrupt_pco=off  eqepinterrupt_pcr=off  eqepinterrupt_pcm=off  eqepinterrupt_sel=off  eqepinterrupt_iel=off  eqepinterrupt_uto=off  pheOutputport=off  watchdogOutputport=off  outport13Datatype=auto  outport14Datatype=auto
  Out : Outport
  wires:
  ADC_C_IN2/1 -> Mux1/1
  Mux1/1 -> Out/1
  ADC_B_IN2/1 -> Mux1/2
  Sim/1 -> Terminator/1
  eQEP/1 -> Mux1/3
  eQEP/2 -> Mux1/4

== system testing/Current Control/HW_Inputs/Sensor Driver Blocks (sim) ==
  Sim : Inport
  Out : Outport
  wires:
  Sim/1 -> Out/1

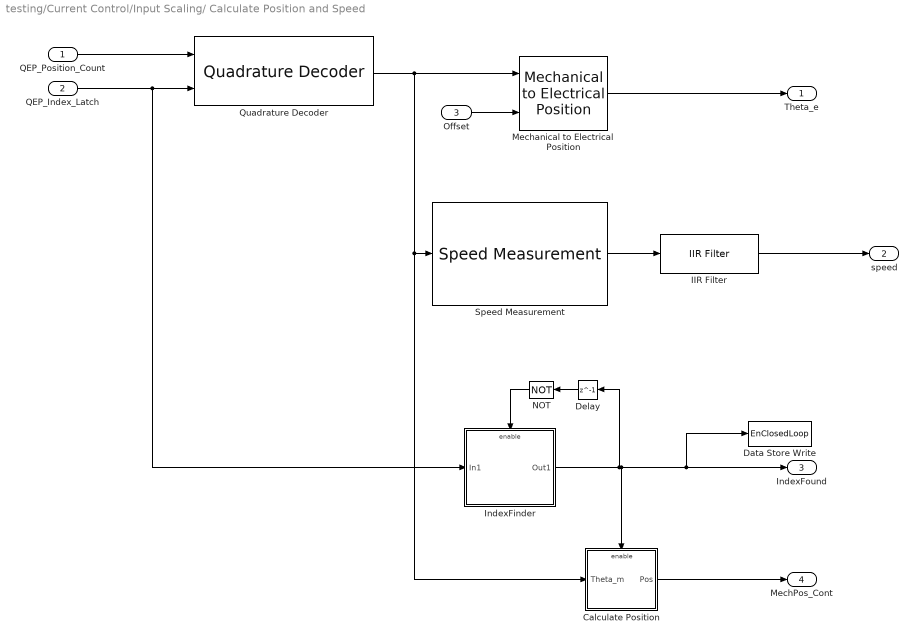
== system testing/Current Control/Input Scaling/ Calculate Position and Speed ==
  QEP_Position_Count : Inport
  QEP_Index_Latch : Inport  Port=2
  Offset : Inport  Port=3
  Calculate Position : Subsystem
  Data Store Write : DataStoreWrite  DataStoreName=EnClosedLoop  IndexOptions=Index vector (dialog)  Indices=1  OutputSizes=1
  Delay : Delay  DelayLength=1
  IIR Filter : mcbcontrolslib/IIR Filter  VariantControl=Low Pass Filter  VariantSelect=Low-pass  FilterConstantInputType=Specify via dialog  Filter_constant=LPFltCoeff  InitialOutput=Specify via dialog  InitialOutputValue=0  ExternalReset=none  advancedSettings=off  Ts=50e-6  cutOff_freq=32.1525
  IndexFinder : Subsystem
  Mechanical to Electrical Position : mcbpositiondecoderlib/Mechanical to Electrical Position  PolePairsInputType=Specify via dialog  NrPP=pmsm.p  selectedRange=Radians  MechOfstInputType=Input port  mechOffsetIn=0  maxAngleIn=2*pi  InputDataType=dataType  VariantSelect=floating-point
  NOT : Logic  Operator=NOT  AllPortsSameDT=off  OutDataTypeStr=boolean
  Quadrature Decoder : mcbpositiondecoderlib/Quadrature Decoder  ParameterInputType=off  CountsPerRevInverseDataType=single  EncoderSlitsPerRevolution=pmsm.QEPSlits  EncoderCountsPerSlit=4  CounterSize=16 bits  ExternalIndexCount=on  PositionUnit=Radians  PositionDataType=dataType
  Speed Measurement : mcbpositiondecoderlib/Speed Measurement  DiscreteStepInput=off  LastDiscreteStepInput=off  PositionUnit=Radians  PositionScalingDatatype=uint32  SpeedCalculationMode=Time interval for speed calculation  TempSpeedCalculationMode=Time interval for speed calculation  SampleTimeAsync=Ts  MaximumApplicationSpeed=6000  SpeedResolution=5e-6  DelayLength=20  MaximumMeasurableSpeed=28571.4286  MeasurableSpeedResolution=1.397e-05  SpeedUnit=Radians/Sec  TempSpeedUnit=RPM  PerUnitSpeed=PU_System.N_base  SpeedDataType=dataType
  Theta_e : Outport  VectorParamsAs1DForOutWhenUnconnected=off
  speed : Outport  Port=2  VectorParamsAs1DForOutWhenUnconnected=off
  IndexFound : Outport  Port=3  InitialOutput=0  VectorParamsAs1DForOutWhenUnconnected=off
  MechPos_Cont : Outport  Port=4  InitialOutput=0  VectorParamsAs1DForOutWhenUnconnected=off
  wires:
  Speed Measurement/1 -> IIR Filter/1
  Mechanical to Electrical Position/1 -> Theta_e/1
  QEP_Position_Count/1 -> Quadrature Decoder/1
  Quadrature Decoder/1 -> Calculate Position/1(Theta_m), Speed Measurement/1, Mechanical to Electrical Position/1
  Offset/1 -> Mechanical to Electrical Position/2
  IIR Filter/1 -> speed/1
  Delay/1 -> NOT/1
  NOT/1 -> IndexFinder/Enable
  IndexFinder/1(Out1) -> Data Store Write/1, IndexFound/1, Calculate Position/Enable, Delay/1
  QEP_Index_Latch/1 -> IndexFinder/1(In1), Quadrature Decoder/2
  Calculate Position/1(Pos) -> MechPos_Cont/1

== system testing/Current Control/Input Scaling/Calculate Phase Currents ==
  Ia_ADC : Inport
  Ib_ADC : Inport  Port=2
  Add : Sum  Inputs=-+
  Data Store Read1 : DataStoreRead  DataStoreName=IaOffset  IndexOptions=Index vector (dialog)  Indices=1  OutputSizes=1
  Data Store Read2 : DataStoreRead  DataStoreName=IbOffset  IndexOptions=Index vector (dialog)  Indices=1  OutputSizes=1
  Data Type Conversion : DataTypeConversion  OutDataTypeStr=int32  ConvertRealWorld=Stored Integer (SI)  RndMeth=Simplest  SaturateOnIntegerOverflow=off
  Get ADC Voltage : Gain  Gain=target.ADC_Vref /target.ADC_MaxCount  OutDataTypeStr=dataType  RndMeth=Simplest
  Get Currents : Gain  Gain=inverter.invertingAmp/inverter.ISenseVoltPerAmp  RndMeth=Simplest  OutDataTypeStr=Inherit: Same as input
  Mux : Mux  Inputs=2
  Mux1 : Mux  Inputs=2
  Iab_meas : Outport  VectorParamsAs1DForOutWhenUnconnected=off
  wires:
  Data Type Conversion/1 -> Add/2
  Ia_ADC/1 -> Mux/1
  Ib_ADC/1 -> Mux/2
  Mux/1 -> Data Type Conversion/1
  Data Store Read1/1 -> Mux1/1
  Data Store Read2/1 -> Mux1/2
  Mux1/1 -> Add/1
  Get Currents/1 -> Iab_meas/1
  Get ADC Voltage/1 -> Get Currents/1
  Add/1 -> Get ADC Voltage/1
